simulink model "ssc_hydromech_power_split_cvt_engine_signal_intf"  (R2025a)
settings: Solver=ode23t  StartTime=0.0  StopTime=70  RelTol=1e-3  AbsTol=1e-3
StartFcn:
  | tic
StopFcn:
  | Elapsed_Sim_Time = toc;
  | disp(['Elapsed Sim Time = ' num2str(Elapsed_Sim_Time)]);
undefined symbols (not defined in the file): DiscIntNeverNeededParam, HMPST, K, Lambda, tau, x0
libraries: fl_lib x30, nesl_utility x16, sm_wheel_loader_lib x9, simulink x7, simulink_extras x6, sdl_lib x3
(part 1 of 4)
Description:
  | Wheel Loader CVT with Signal Interface
  | Copyright 2023-2025 The MathWorks, Inc.
settings Model: TunableVars=Init_Veh_TopSpeed  TunableVarsStorageClass=Auto  Creator=Shusen Zhang  LastModifiedBy=smiller
settings SolverCC: AutoScaleAbsTol=off  MaxConsecutiveMinStep=5
settings DataIOCC: ReturnWorkspaceOutputs=off  SignalLoggingName=logsout_ssc_hydromech_power_split_cvt_engine_signal_intf
settings DebuggingCC: UnderspecifiedInitializationDetection=Classic  MergeDetectMultiDrivingBlocksExec=none
settings ModelReferenceCC: PropagateSignalLabelsOutOfModel=off
settings RTWCC: GPUComputeCapability=3.5
settings SimscapeCC: SimscapeLogType=all  SimscapeLogName=simlog_ssc_hydromech_power_split_cvt_engine_signal_intf  SimscapeLogLimitData=off
settings ExplorerConfigSet: SimMechanicsOpenEditorOnUpdate=off

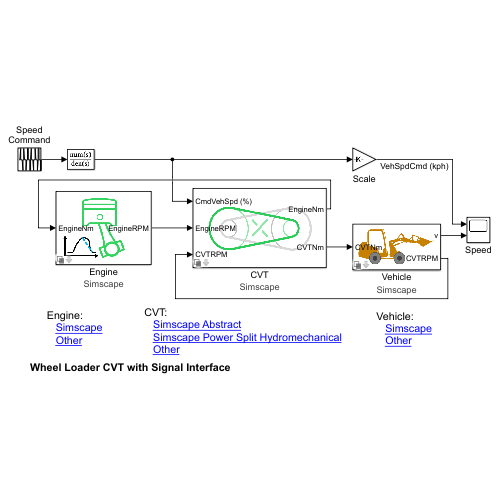
[thumbnail: Simulink's stored preview of the top-level diagram]
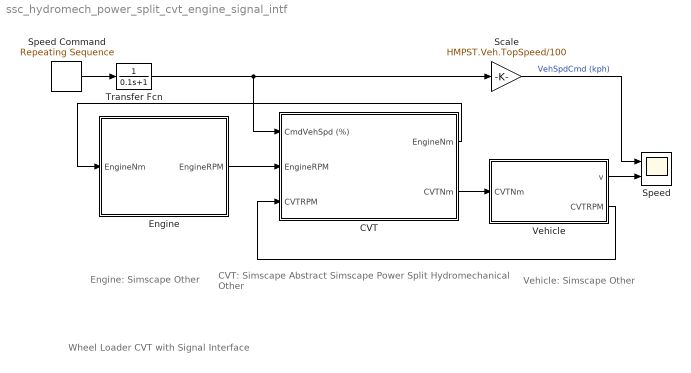
== system ssc_hydromech_power_split_cvt_engine_signal_intf ==
  note: Wheel Loader CVT with Signal Interface
  note: CVT:
      | Simscape Abstract
      | Simscape Power Split Hydromechanical
      | Other
  note: Vehicle:
      | Simscape
      | Other
  note: Engine:
      | Simscape
      | Other
  CVT : Subsystem  Variant=on  VariantControlMode=label  VariantControl=CVT  LabelModeActiveChoice=Simscape
      settings: AttributesFormatString=%<LabelModeActiveChoice>
  Engine : Subsystem  Variant=on  VariantControlMode=label  VariantControl=Engine  LabelModeActiveChoice=Simscape
      settings: AttributesFormatString=%<LabelModeActiveChoice>
  Scale : Gain  Gain=HMPST.Veh.TopSpeed/100
  Speed : Scope  NumInputPorts=2
      settings: ActiveDisplayYMinimum=-9.8692  ActiveDisplayYMaximum=9.88206
  Speed Command : simulink/Sources/Repeating Sequence  rep_seq_t=[0 10 12 15 17 32 34 37 39 41 43 46 48 63 65 68 70]  rep_seq_y=[0 0 1 1 0 0 -1 -1 0 0 1 1 0 0 -1 -1 0]*25
  Transfer Fcn : TransferFcn  Denominator=[0.1 1]
  Vehicle : Subsystem  Variant=on  VariantControlMode=label  VariantControl=Vehicle  LabelModeActiveChoice=Simscape
      settings: AttributesFormatString=%<LabelModeActiveChoice>
  wires:
  Speed Command/1 -> Transfer Fcn/1
  Transfer Fcn/1 -> Scale/1, CVT/1(CmdVehSpd (%))
  Engine/1(EngineRPM) -> CVT/2(EngineRPM)
  CVT/1(EngineNm) -> Engine/1(EngineNm)
  CVT/2(CVTNm) -> Vehicle/1(CVTNm)
  Vehicle/1(v) -> Speed/2
  Vehicle/2(CVTRPM) -> CVT/3(CVTRPM)
  Scale/1 -> Speed/1  "VehSpdCmd (kph)"

== system ssc_hydromech_power_split_cvt_engine_signal_intf/CVT ==
  CmdVehSpd (%) : Inport
  EngineRPM : Inport  Port=2
  CVTRPM : Inport  Port=3
  Other : Subsystem  VariantControl=Other
  Simscape : Subsystem  VariantControl=Simscape
      mask Display:
      | activeVar = get_param([gcb '/Transmission'],'LabelModeActiveChoice');
      | 
      | if(strcmp(activeVar,'Abstract'))
      |     image('ssc_cvt_abstract_IMAGE.png');
      | elseif(strcmp(activeVar,'Hydrostatic'))
      |     image('sm_wheel_loader_hydrostatic_IMAGE.png');
      | elseif(strcmp(activeVar,'Power_Split_HM'))
      |     image('ssc_hydromech_power_split_cvt_IMAGE.png');
      | end
  EngineNm : Outport
  CVTNm : Outport  Port=2

== system ssc_hydromech_power_split_cvt_engine_signal_intf/Engine ==
  EngineNm : Inport
  Other : Subsystem  VariantControl=Other
  Simscape : Subsystem  VariantControl=Simscape
      mask Display: image('sdl_engine_Droop_IMAGE.png')
  EngineRPM : Outport

== system ssc_hydromech_power_split_cvt_engine_signal_intf/Vehicle ==
  CVTNm : Inport
  Other : Subsystem  VariantControl=Other
  Simscape : Subsystem  VariantControl=Simscape
      mask Display: image('sm_wheel_loader_vehicle1D_IMAGE.png');
  v : Outport
  CVTRPM : Outport  Port=2

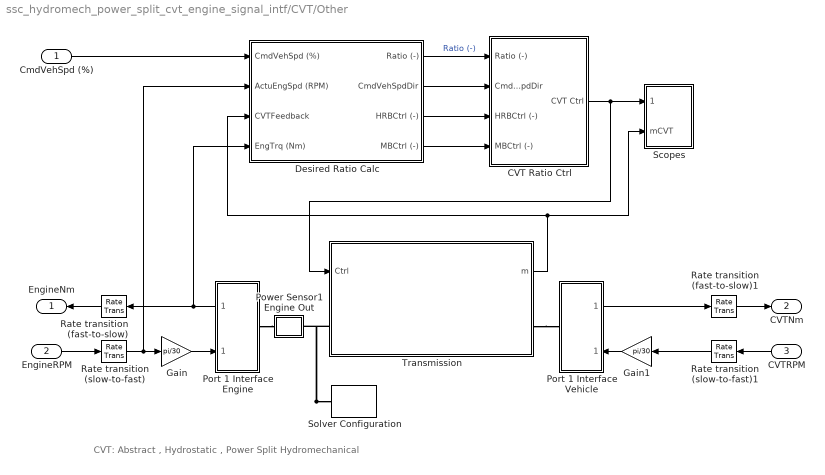
== system ssc_hydromech_power_split_cvt_engine_signal_intf/CVT/Other ==
  note: CVT: Abstract , Hydrostatic , Power Split Hydromechanical
  CmdVehSpd (%) : Inport
  EngineRPM : Inport  Port=2
  CVTRPM : Inport  Port=3
  CVT Ratio Ctrl : Subsystem
  Desired Ratio Calc : Subsystem
  Gain : Gain  Gain=pi/30
  Gain1 : Gain  Gain=pi/30
  Port 1 Interface Engine : Subsystem  mask(Network Coupler (Flexible Shaft) Port 1 Interface){interfaceModel=an actual shaft compliance, k=250, lambda=20*10, samplingType=Variable step at port 1 and fixed step at port 2, ts=0.001, h1=0.001, h2=1/60, predictionDiscreteToContinuous=off, smoothingContinuousToDiscrete=off, predictionSlowToFast=off, smoothingFastToSlow=off, nSmooth=1, tsSmoothing=0.01, J1=1, J2=1, tsRecommended=0.0026611, hRecommended=0.00026611, kDerived=250, lambdaDerived=20, tsMax=0.11975, through0=0}
      mask prompts: interfaceModel "physmod:simscape:couplers:SimscapeNetworkCouplersLib:SeparateUsing_MP"; k "physmod:simscape:couplers:SimscapeNetworkCouplersLib:ShaftStiffnessNmrad_MP"; lambda "physmod:simscape:couplers:SimscapeNetworkCouplersLib:ShaftDampingNmrads_MP"; samplingType "physmod:simscape:couplers:SimscapeNetworkCouplersLib:SamplingType_MP"; ts "physmod:simscape:couplers:SimscapeNetworkCouplersLib:SeparatorTimeConstants_MP"; h1 "physmod:simscape:couplers:SimscapeNetworkCouplersLib:Port1NetworkDiscreteSampleTimes_MP"; h2 "physmod:simscape:couplers:SimscapeNetworkCouplersLib:Port2NetworkDiscreteSampleTimes_MP"; predictionDiscreteToContinuous "physmod:simscape:couplers:SimscapeNetworkCouplersLib:UsePredictionWhenConnectingFixedStepToVariableStep_MP"; smoothingContinuousToDiscrete "physmod:simscape:couplers:SimscapeNetworkCouplersLib:UseSmoothingWhenConnectingVariableStepToFixedStep_MP"; predictionSlowToFast "physmod:simscape:couplers:SimscapeNetworkCouplersLib:UsePredictionWhenConnectingSlowToFastSampleTimes_MP"; smoothingFastToSlow "physmod:simscape:couplers:SimscapeNetworkCouplersLib:UseSmoothingWhenConnectingFastToSlowSampleTimes_MP"; nSmooth "physmod:simscape:couplers:SimscapeNetworkCouplersLib:NumberOfSamplesOverWhichToSmooth_MP"; tsSmoothing "physmod:simscape:couplers:SimscapeNetworkCouplersLib:SmoothingTimeConstants_MP"; J1 "physmod:simscape:couplers:SimscapeNetworkCouplersLib:ApproximateInertiaAtPort1kgm2_MP"; J2 "physmod:simscape:couplers:SimscapeNetworkCouplersLib:ApproximateInertiaAtPort2kgm2_MP"; tsRecommended "physmod:simscape:couplers:SimscapeNetworkCouplersLib:RecommendedMaxFilterTimeConstants_MP"; hRecommended "physmod:simscape:couplers:SimscapeNetworkCouplersLib:RecommendedMaxDiscreteSampleTimes_MP"; kDerived "physmod:simscape:couplers:SimscapeNetworkCouplersLib:CalculatedShaftStiffnessNmrad_MP"; lambdaDerived "physmod:simscape:couplers:SimscapeNetworkCouplersLib:CalculatedShaftDampingNmrads_MP"; tsMax "physmod:simscape:couplers:SimscapeNetworkCouplersLib:CalculatedFastestTrackableTimeConstants_MP"; through0 "physmod:simscape:couplers:SimscapeNetworkCouplersLib:InitialTransmittedTorqueNm_MP"
      mask help: physmod:simscape:couplers:SimscapeNetworkCouplersLib:NetworkCouplerFlexibleShaftPort1Interface_MD
      mask init:
      | % Fixed step sample time value check
      | foundation.internal.couplers.checkSampleTimes(gcb,h1,h2);
      | 
      | % Map mask choices to Simscape block parameters  
      | [K,Lambda,tau,~,~,x0,~] = foundation.internal.couplers.mechanical.derivedParamsRotational(...
      |     gcb,ts,h1,h2,through0,k,lambda,J1,J2);
      settings: PortSchema="{\"entries\":[{\"content\":{\"sides\":[{\"content\":{\"connectorIds\":[\"LConn1\"]},\"type\":\"ConnectorPlacement.EquallySpacedRectSide\",\"uuid\":\"a6d4a9fd-b5aa-40dc-ab7e-2b646b9b57bc\"},{\"content\":{\"connectorIds\":[\"Out1\",\"In1\"],\"side\":\"RIGHT\"},\"type\":\"ConnectorPlacement.EquallySpacedRectSide\",\"uuid\":\"31bb6273-5b9b-48d0-a1a2-6fbacb979b97\"},{\"content\":{\"connectorIds\":[],\"side\":\"TOP\"},\"type\":\"ConnectorPlacement.EquallySpacedRectSide\",\"uuid\":\"0f7afab2-4481-486c-9ad0-2b42c5b091a4\"}]},\"type\":\"ConnectorPlacement.EquallySpacedConnector\",\"uuid\":\"a98e47aa-cbfd-441a-b14c-c9ea515c056e\"}],\"packageUris\":[\"http://schema.mathworks.com/mf0/Connector/R2020b\"],\"version\":\"1.0\"}"
      mask Help: web([docroot '/simscape/ref/networkcouplerflexibleshaft.html'])
      mask TypeOptions interfaceModel: physmod:simscape:couplers:SimscapeNetworkCouplersLib:anActualShaftCompliance_PV | physmod:simscape:couplers:SimscapeNetworkCouplersLib:anAddedNumericalCompliance_PV
      mask Callback interfaceModel: foundation.internal.couplers.mechanical.parameterVisibilities(gcb)
      mask TypeOptions samplingType: physmod:simscape:couplers:SimscapeNetworkCouplersLib:VariableStepAtPorts1And2_PV | physmod:simscape:couplers:SimscapeNetworkCouplersLib:VariableStepAtPort1AndFixedStepAtPort2_PV | physmod:simscape:couplers:SimscapeNetworkCouplersLib:FixedStepBothPortsWithCommonSampleTime_PV | physmod:simscape:couplers:SimscapeNetworkCouplersLib:FixedStepBothPortsWithFasterSamplingAtPort1_PV
      mask Callback samplingType: foundation.internal.couplers.mechanical.parameterVisibilities(gcb)
      mask Callback predictionDiscreteToContinuous: foundation.internal.couplers.mechanical.parameterVisibilities(gcb)
      mask Callback smoothingContinuousToDiscrete: foundation.internal.couplers.mechanical.parameterVisibilities(gcb)
      mask Callback predictionSlowToFast: foundation.internal.couplers.mechanical.parameterVisibilities(gcb)
      mask Callback smoothingFastToSlow: foundation.internal.couplers.mechanical.parameterVisibilities(gcb)
      mask DialogControl Main Prompt: physmod:simscape:couplers:SimscapeNetworkCouplersLib:tab_Main
      mask DialogControl interfaceModel Prompt: Separate using
      mask DialogControl k Prompt: Shaft stiffness (Nm/rad)
      mask DialogControl lambda Prompt: Shaft damping (Nm/(rad/s))
      mask DialogControl samplingType Prompt: Sampling type
      mask DialogControl ts Prompt: Separator time constant (s)
      mask DialogControl h1 Prompt: Port 1 network discrete sample time (s)
      mask DialogControl h2 Prompt: Port 2 network discrete sample time (s)
      mask DialogControl predictionDiscreteToContinuous Prompt: Use prediction when connecting fixed step to variable step
      mask DialogControl smoothingContinuousToDiscrete Prompt: Use smoothing when connecting variable step to fixed step
      mask DialogControl predictionSlowToFast Prompt: Use prediction when connecting slow to fast sample times
      mask DialogControl smoothingFastToSlow Prompt: Use smoothing when connecting fast to slow sample times
      mask DialogControl nSmooth Prompt: Number of samples over which to smooth
      mask DialogControl tsSmoothing Prompt: Smoothing time constant (s)
      mask DialogControl Analysis Prompt: physmod:simscape:couplers:SimscapeNetworkCouplersLib:tab_Analysis
      mask DialogControl connectedNetworkInfo Prompt: physmod:simscape:couplers:SimscapeNetworkCouplersLib:heading_ConnectedNetworkInformation
      mask DialogControl J1 Prompt: Approximate inertia at port 1 (kg*m^2)
      mask DialogControl J2 Prompt: Approximate inertia at port 2 (kg*m^2)
      mask DialogControl derivedValues Prompt: physmod:simscape:couplers:SimscapeNetworkCouplersLib:heading_DerivedValues
      mask DialogControl tsRecommended Prompt: Recommended max filter time constant (s)
      mask DialogControl hRecommended Prompt: Recommended max discrete sample time (s)
      mask DialogControl kDerived Prompt: Calculated shaft stiffness (Nm/rad)
      mask DialogControl lambdaDerived Prompt: Calculated shaft damping (Nm/(rad/s))
      mask DialogControl tsMax Prompt: Calculated fastest trackable time constant (s)
      mask DialogControl updateRecommendations Prompt: physmod:simscape:couplers:SimscapeNetworkCouplersLib:button_Update
      mask DialogControl updateRecommendations Callback: foundation.internal.couplers.mechanical.analysisRotational(gcb);
      mask DialogControl InitialConditions Prompt: physmod:simscape:couplers:SimscapeNetworkCouplersLib:tab_InitialConditions
      mask DialogControl through0 Prompt: Initial transmitted torque (Nm)
  Port 1 Interface Vehicle : Subsystem  mask(Network Coupler (Flexible Shaft) Port 1 Interface){interfaceModel=an actual shaft compliance, k=250*10, lambda=20*10, samplingType=Variable step at port 1 and fixed step at port 2, ts=0.001, h1=0.001, h2=1/60, predictionDiscreteToContinuous=off, smoothingContinuousToDiscrete=off, predictionSlowToFast=off, smoothingFastToSlow=off, nSmooth=1, tsSmoothing=0.01, J1=1, J2=1, tsRecommended=0.0026611, hRecommended=0.00026611, kDerived=250, lambdaDerived=20, tsMax=0.11975, through0=0}
      mask prompts: interfaceModel "physmod:simscape:couplers:SimscapeNetworkCouplersLib:SeparateUsing_MP"; k "physmod:simscape:couplers:SimscapeNetworkCouplersLib:ShaftStiffnessNmrad_MP"; lambda "physmod:simscape:couplers:SimscapeNetworkCouplersLib:ShaftDampingNmrads_MP"; samplingType "physmod:simscape:couplers:SimscapeNetworkCouplersLib:SamplingType_MP"; ts "physmod:simscape:couplers:SimscapeNetworkCouplersLib:SeparatorTimeConstants_MP"; h1 "physmod:simscape:couplers:SimscapeNetworkCouplersLib:Port1NetworkDiscreteSampleTimes_MP"; h2 "physmod:simscape:couplers:SimscapeNetworkCouplersLib:Port2NetworkDiscreteSampleTimes_MP"; predictionDiscreteToContinuous "physmod:simscape:couplers:SimscapeNetworkCouplersLib:UsePredictionWhenConnectingFixedStepToVariableStep_MP"; smoothingContinuousToDiscrete "physmod:simscape:couplers:SimscapeNetworkCouplersLib:UseSmoothingWhenConnectingVariableStepToFixedStep_MP"; predictionSlowToFast "physmod:simscape:couplers:SimscapeNetworkCouplersLib:UsePredictionWhenConnectingSlowToFastSampleTimes_MP"; smoothingFastToSlow "physmod:simscape:couplers:SimscapeNetworkCouplersLib:UseSmoothingWhenConnectingFastToSlowSampleTimes_MP"; nSmooth "physmod:simscape:couplers:SimscapeNetworkCouplersLib:NumberOfSamplesOverWhichToSmooth_MP"; tsSmoothing "physmod:simscape:couplers:SimscapeNetworkCouplersLib:SmoothingTimeConstants_MP"; J1 "physmod:simscape:couplers:SimscapeNetworkCouplersLib:ApproximateInertiaAtPort1kgm2_MP"; J2 "physmod:simscape:couplers:SimscapeNetworkCouplersLib:ApproximateInertiaAtPort2kgm2_MP"; tsRecommended "physmod:simscape:couplers:SimscapeNetworkCouplersLib:RecommendedMaxFilterTimeConstants_MP"; hRecommended "physmod:simscape:couplers:SimscapeNetworkCouplersLib:RecommendedMaxDiscreteSampleTimes_MP"; kDerived "physmod:simscape:couplers:SimscapeNetworkCouplersLib:CalculatedShaftStiffnessNmrad_MP"; lambdaDerived "physmod:simscape:couplers:SimscapeNetworkCouplersLib:CalculatedShaftDampingNmrads_MP"; tsMax "physmod:simscape:couplers:SimscapeNetworkCouplersLib:CalculatedFastestTrackableTimeConstants_MP"; through0 "physmod:simscape:couplers:SimscapeNetworkCouplersLib:InitialTransmittedTorqueNm_MP"
      mask help: physmod:simscape:couplers:SimscapeNetworkCouplersLib:NetworkCouplerFlexibleShaftPort1Interface_MD
      mask init: same as ssc_hydromech_power_split_cvt_engine_signal_intf/CVT/Other/Port 1 Interface Engine
      settings: PortSchema="{\"entries\":[{\"content\":{\"sides\":[{\"content\":{\"connectorIds\":[\"LConn1\"]},\"type\":\"ConnectorPlacement.EquallySpacedRectSide\",\"uuid\":\"a6d4a9fd-b5aa-40dc-ab7e-2b646b9b57bc\"},{\"content\":{\"connectorIds\":[\"Out1\",\"In1\"],\"side\":\"RIGHT\"},\"type\":\"ConnectorPlacement.EquallySpacedRectSide\",\"uuid\":\"31bb6273-5b9b-48d0-a1a2-6fbacb979b97\"},{\"content\":{\"connectorIds\":[],\"side\":\"TOP\"},\"type\":\"ConnectorPlacement.EquallySpacedRectSide\",\"uuid\":\"0f7afab2-4481-486c-9ad0-2b42c5b091a4\"}]},\"type\":\"ConnectorPlacement.EquallySpacedConnector\",\"uuid\":\"a98e47aa-cbfd-441a-b14c-c9ea515c056e\"}],\"packageUris\":[\"http://schema.mathworks.com/mf0/Connector/R2020b\"],\"version\":\"1.0\"}"
      mask Help: web([docroot '/simscape/ref/networkcouplerflexibleshaft.html'])
      mask TypeOptions interfaceModel: physmod:simscape:couplers:SimscapeNetworkCouplersLib:anActualShaftCompliance_PV | physmod:simscape:couplers:SimscapeNetworkCouplersLib:anAddedNumericalCompliance_PV
      mask Callback interfaceModel: foundation.internal.couplers.mechanical.parameterVisibilities(gcb)
      mask TypeOptions samplingType: physmod:simscape:couplers:SimscapeNetworkCouplersLib:VariableStepAtPorts1And2_PV | physmod:simscape:couplers:SimscapeNetworkCouplersLib:VariableStepAtPort1AndFixedStepAtPort2_PV | physmod:simscape:couplers:SimscapeNetworkCouplersLib:FixedStepBothPortsWithCommonSampleTime_PV | physmod:simscape:couplers:SimscapeNetworkCouplersLib:FixedStepBothPortsWithFasterSamplingAtPort1_PV
      mask Callback samplingType: foundation.internal.couplers.mechanical.parameterVisibilities(gcb)
      mask Callback predictionDiscreteToContinuous: foundation.internal.couplers.mechanical.parameterVisibilities(gcb)
      mask Callback smoothingContinuousToDiscrete: foundation.internal.couplers.mechanical.parameterVisibilities(gcb)
      mask Callback predictionSlowToFast: foundation.internal.couplers.mechanical.parameterVisibilities(gcb)
      mask Callback smoothingFastToSlow: foundation.internal.couplers.mechanical.parameterVisibilities(gcb)
      mask DialogControl Main Prompt: physmod:simscape:couplers:SimscapeNetworkCouplersLib:tab_Main
      mask DialogControl interfaceModel Prompt: Separate using
      mask DialogControl k Prompt: Shaft stiffness (Nm/rad)
      mask DialogControl lambda Prompt: Shaft damping (Nm/(rad/s))
      mask DialogControl samplingType Prompt: Sampling type
      mask DialogControl ts Prompt: Separator time constant (s)
      mask DialogControl h1 Prompt: Port 1 network discrete sample time (s)
      mask DialogControl h2 Prompt: Port 2 network discrete sample time (s)
      mask DialogControl predictionDiscreteToContinuous Prompt: Use prediction when connecting fixed step to variable step
      mask DialogControl smoothingContinuousToDiscrete Prompt: Use smoothing when connecting variable step to fixed step
      mask DialogControl predictionSlowToFast Prompt: Use prediction when connecting slow to fast sample times
      mask DialogControl smoothingFastToSlow Prompt: Use smoothing when connecting fast to slow sample times
      mask DialogControl nSmooth Prompt: Number of samples over which to smooth
      mask DialogControl tsSmoothing Prompt: Smoothing time constant (s)
      mask DialogControl Analysis Prompt: physmod:simscape:couplers:SimscapeNetworkCouplersLib:tab_Analysis
      mask DialogControl connectedNetworkInfo Prompt: physmod:simscape:couplers:SimscapeNetworkCouplersLib:heading_ConnectedNetworkInformation
      mask DialogControl J1 Prompt: Approximate inertia at port 1 (kg*m^2)
      mask DialogControl J2 Prompt: Approximate inertia at port 2 (kg*m^2)
      mask DialogControl derivedValues Prompt: physmod:simscape:couplers:SimscapeNetworkCouplersLib:heading_DerivedValues
      mask DialogControl tsRecommended Prompt: Recommended max filter time constant (s)
      mask DialogControl hRecommended Prompt: Recommended max discrete sample time (s)
      mask DialogControl kDerived Prompt: Calculated shaft stiffness (Nm/rad)
      mask DialogControl lambdaDerived Prompt: Calculated shaft damping (Nm/(rad/s))
      mask DialogControl tsMax Prompt: Calculated fastest trackable time constant (s)
      mask DialogControl updateRecommendations Prompt: physmod:simscape:couplers:SimscapeNetworkCouplersLib:button_Update
      mask DialogControl updateRecommendations Callback: foundation.internal.couplers.mechanical.analysisRotational(gcb);
      mask DialogControl InitialConditions Prompt: physmod:simscape:couplers:SimscapeNetworkCouplersLib:tab_InitialConditions
      mask DialogControl through0 Prompt: Initial transmitted torque (Nm)
  Power Sensor1 Engine Out : Subsystem
  Rate transition (fast-to-slow) : RateTransition  Integrity=off
  Rate transition (fast-to-slow)1 : RateTransition  Integrity=off
  Rate transition (slow-to-fast) : RateTransition  Integrity=off
  Rate transition (slow-to-fast)1 : RateTransition  Integrity=off
  Scopes : Subsystem
  Solver Configuration : nesl_utility/Solver Configuration  PhysicalDomain=network_engine_domain  SubClassName=solver  LeftPortType=input  RightPortType=generic  Tones=[]  Harmonics=[]  SimulateNoise=off  Profile=off  UseLocalSampling=off  EnableSwitchedLinearOptims=on  FrequencyDomain=off  UseCCode=off  RelTol=0.001  AbsTol=1e-06  MinStep=1e-09  ToWorkspace=off  RevertToSquareIcSolve=off  NumHomotopyIterations=100  PhasorMode=off  PhasorModeNumHarmonics=1  ConsistencySolver=NEWTON_XTOL_AFTER_FTOL  IndexReductionMethod=DerivativeReplacement  DoDC=off  ResidualTolerance=1e-09  ConsistencyTolSource=GLOBAL  ConsistencyAbsTol=0.001  ConsistencyRelTol=0.001  ConsistencyTolFactor=0.001  UseLocalSolver=off  LocalSolverChoice=NE_BACKWARD_EULER_ADVANCER  ResolveIndetEquations=on  FunctionEvalNumThread=1  LocalSolverSampleTime=0.001  DoFixedCost=off  MaxNonlinIter=1  MaxModeIter=2  ComputeImpulses=off  ImpulseIterations=2  LinearAlgebra=Sparse  LinearAlgebraNumThread=0  EquationFormulation=NE_TIME_EF  DelaysMemoryBudget=1024  AutomaticFiltering=on  FilteringTimeConstant=0.001  PartitionStorageMethod=AS_NEEDED  PartitionMemoryBudget=1024  PartitionMethod=FAST  MultibodyUseLocalSolver=off  MultibodyLocalSolverChoice=ODE1  MultibodyLocalSolverSampleTime=0.001
  Transmission : Subsystem  Variant=on  VariantControlMode=label  VariantControl=Choice  LabelModeActiveChoice=Abstract
      settings: AttributesFormatString=%<LabelModeActiveChoice>
  EngineNm : Outport
  CVTNm : Outport  Port=2
  wires:
  Transmission/1(m) -> Desired Ratio Calc/3(CVTFeedback), Scopes/2(mCVT)
  CVT Ratio Ctrl/1(CVT Ctrl) -> Scopes/1(CVTCtrl), Transmission/1(Ctrl)
  EngineRPM/1 -> Rate transition (slow-to-fast)/1
  Rate transition (slow-to-fast)1/1 -> Gain1/1
  Port 1 Interface Vehicle/1(torque) -> Rate transition (fast-to-slow)1/1
  CVTRPM/1 -> Rate transition (slow-to-fast)1/1
  Gain/1 -> Port 1 Interface Engine/1(speed)
  Gain1/1 -> Port 1 Interface Vehicle/1(speed)
  Rate transition (fast-to-slow)1/1 -> CVTNm/1
  Rate transition (fast-to-slow)/1 -> EngineNm/1
  CmdVehSpd (%)/1 -> Desired Ratio Calc/1(CmdVehSpd (%))
  Desired Ratio Calc/4(MBCtrl (-)) -> CVT Ratio Ctrl/4(MBCtrl (-))
  Rate transition (slow-to-fast)/1 -> Gain/1, Desired Ratio Calc/2(ActuEngSpd (RPM))
  Port 1 Interface Engine/1(torque) -> Rate transition (fast-to-slow)/1, Desired Ratio Calc/4(EngTrq (Nm))
  Desired Ratio Calc/1(Ratio (-)) -> CVT Ratio Ctrl/1(Ratio (-))  "Ratio (-)"
  Desired Ratio Calc/2(CmdVehSpdDir) -> CVT Ratio Ctrl/2(CmdVehSpdDir)
  Desired Ratio Calc/3(HRBCtrl (-)) -> CVT Ratio Ctrl/3(HRBCtrl (-))
  connections:
  Solver Configuration/RConn1 -- Transmission/LConn1 -- Power Sensor1 Engine Out/RConn1
  Port 1 Interface Engine/LConn1 -- Power Sensor1 Engine Out/LConn1
  Transmission/RConn1 -- Port 1 Interface Vehicle/LConn1

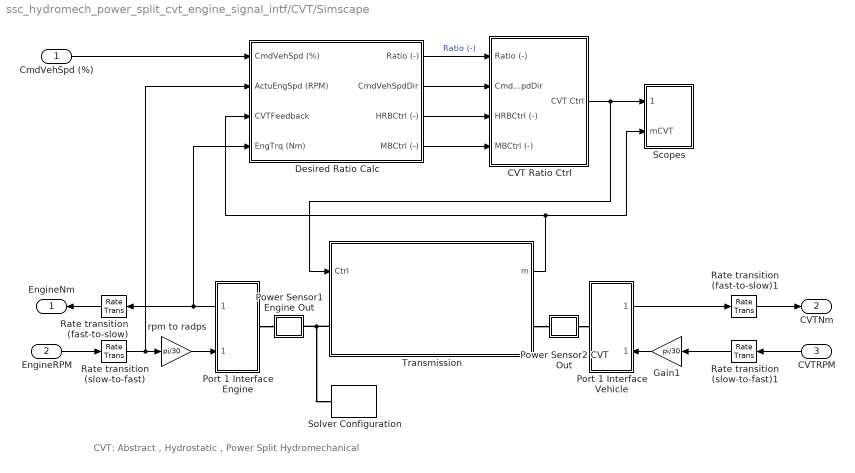
== system ssc_hydromech_power_split_cvt_engine_signal_intf/CVT/Simscape ==
  note: CVT: Abstract , Hydrostatic , Power Split Hydromechanical
  CmdVehSpd (%) : Inport
  EngineRPM : Inport  Port=2
  CVTRPM : Inport  Port=3
  CVT Ratio Ctrl : Subsystem
  Desired Ratio Calc : Subsystem
  Gain1 : Gain  Gain=pi/30
  Port 1 Interface Engine : Subsystem  mask(Network Coupler (Flexible Shaft) Port 1 Interface){interfaceModel=an actual shaft compliance, k=250, lambda=20*10, samplingType=Variable step at port 1 and fixed step at port 2, ts=0.001, h1=0.001, h2=1/60, predictionDiscreteToContinuous=off, smoothingContinuousToDiscrete=off, predictionSlowToFast=off, smoothingFastToSlow=off, nSmooth=1, tsSmoothing=0.01, J1=1, J2=1, tsRecommended=0.0026611, hRecommended=0.00026611, kDerived=250, lambdaDerived=20, tsMax=0.11975, through0=70}
      mask prompts: interfaceModel "physmod:simscape:couplers:SimscapeNetworkCouplersLib:SeparateUsing_MP"; k "physmod:simscape:couplers:SimscapeNetworkCouplersLib:ShaftStiffnessNmrad_MP"; lambda "physmod:simscape:couplers:SimscapeNetworkCouplersLib:ShaftDampingNmrads_MP"; samplingType "physmod:simscape:couplers:SimscapeNetworkCouplersLib:SamplingType_MP"; ts "physmod:simscape:couplers:SimscapeNetworkCouplersLib:SeparatorTimeConstants_MP"; h1 "physmod:simscape:couplers:SimscapeNetworkCouplersLib:Port1NetworkDiscreteSampleTimes_MP"; h2 "physmod:simscape:couplers:SimscapeNetworkCouplersLib:Port2NetworkDiscreteSampleTimes_MP"; predictionDiscreteToContinuous "physmod:simscape:couplers:SimscapeNetworkCouplersLib:UsePredictionWhenConnectingFixedStepToVariableStep_MP"; smoothingContinuousToDiscrete "physmod:simscape:couplers:SimscapeNetworkCouplersLib:UseSmoothingWhenConnectingVariableStepToFixedStep_MP"; predictionSlowToFast "physmod:simscape:couplers:SimscapeNetworkCouplersLib:UsePredictionWhenConnectingSlowToFastSampleTimes_MP"; smoothingFastToSlow "physmod:simscape:couplers:SimscapeNetworkCouplersLib:UseSmoothingWhenConnectingFastToSlowSampleTimes_MP"; nSmooth "physmod:simscape:couplers:SimscapeNetworkCouplersLib:NumberOfSamplesOverWhichToSmooth_MP"; tsSmoothing "physmod:simscape:couplers:SimscapeNetworkCouplersLib:SmoothingTimeConstants_MP"; J1 "physmod:simscape:couplers:SimscapeNetworkCouplersLib:ApproximateInertiaAtPort1kgm2_MP"; J2 "physmod:simscape:couplers:SimscapeNetworkCouplersLib:ApproximateInertiaAtPort2kgm2_MP"; tsRecommended "physmod:simscape:couplers:SimscapeNetworkCouplersLib:RecommendedMaxFilterTimeConstants_MP"; hRecommended "physmod:simscape:couplers:SimscapeNetworkCouplersLib:RecommendedMaxDiscreteSampleTimes_MP"; kDerived "physmod:simscape:couplers:SimscapeNetworkCouplersLib:CalculatedShaftStiffnessNmrad_MP"; lambdaDerived "physmod:simscape:couplers:SimscapeNetworkCouplersLib:CalculatedShaftDampingNmrads_MP"; tsMax "physmod:simscape:couplers:SimscapeNetworkCouplersLib:CalculatedFastestTrackableTimeConstants_MP"; through0 "physmod:simscape:couplers:SimscapeNetworkCouplersLib:InitialTransmittedTorqueNm_MP"
      mask help: physmod:simscape:couplers:SimscapeNetworkCouplersLib:NetworkCouplerFlexibleShaftPort1Interface_MD
      mask init: same as ssc_hydromech_power_split_cvt_engine_signal_intf/CVT/Other/Port 1 Interface Engine
      settings: PortSchema="{\"entries\":[{\"content\":{\"sides\":[{\"content\":{\"connectorIds\":[\"LConn1\"]},\"type\":\"ConnectorPlacement.EquallySpacedRectSide\",\"uuid\":\"a6d4a9fd-b5aa-40dc-ab7e-2b646b9b57bc\"},{\"content\":{\"connectorIds\":[\"Out1\",\"In1\"],\"side\":\"RIGHT\"},\"type\":\"ConnectorPlacement.EquallySpacedRectSide\",\"uuid\":\"31bb6273-5b9b-48d0-a1a2-6fbacb979b97\"},{\"content\":{\"connectorIds\":[],\"side\":\"TOP\"},\"type\":\"ConnectorPlacement.EquallySpacedRectSide\",\"uuid\":\"0f7afab2-4481-486c-9ad0-2b42c5b091a4\"}]},\"type\":\"ConnectorPlacement.EquallySpacedConnector\",\"uuid\":\"a98e47aa-cbfd-441a-b14c-c9ea515c056e\"}],\"packageUris\":[\"http://schema.mathworks.com/mf0/Connector/R2020b\"],\"version\":\"1.0\"}"
      mask Help: web([docroot '/simscape/ref/networkcouplerflexibleshaft.html'])
      mask TypeOptions interfaceModel: physmod:simscape:couplers:SimscapeNetworkCouplersLib:anActualShaftCompliance_PV | physmod:simscape:couplers:SimscapeNetworkCouplersLib:anAddedNumericalCompliance_PV
      mask Callback interfaceModel: foundation.internal.couplers.mechanical.parameterVisibilities(gcb)
      mask TypeOptions samplingType: physmod:simscape:couplers:SimscapeNetworkCouplersLib:VariableStepAtPorts1And2_PV | physmod:simscape:couplers:SimscapeNetworkCouplersLib:VariableStepAtPort1AndFixedStepAtPort2_PV | physmod:simscape:couplers:SimscapeNetworkCouplersLib:FixedStepBothPortsWithCommonSampleTime_PV | physmod:simscape:couplers:SimscapeNetworkCouplersLib:FixedStepBothPortsWithFasterSamplingAtPort1_PV
      mask Callback samplingType: foundation.internal.couplers.mechanical.parameterVisibilities(gcb)
      mask Callback predictionDiscreteToContinuous: foundation.internal.couplers.mechanical.parameterVisibilities(gcb)
      mask Callback smoothingContinuousToDiscrete: foundation.internal.couplers.mechanical.parameterVisibilities(gcb)
      mask Callback predictionSlowToFast: foundation.internal.couplers.mechanical.parameterVisibilities(gcb)
      mask Callback smoothingFastToSlow: foundation.internal.couplers.mechanical.parameterVisibilities(gcb)
      mask DialogControl Main Prompt: physmod:simscape:couplers:SimscapeNetworkCouplersLib:tab_Main
      mask DialogControl interfaceModel Prompt: Separate using
      mask DialogControl k Prompt: Shaft stiffness (Nm/rad)
      mask DialogControl lambda Prompt: Shaft damping (Nm/(rad/s))
      mask DialogControl samplingType Prompt: Sampling type
      mask DialogControl ts Prompt: Separator time constant (s)
      mask DialogControl h1 Prompt: Port 1 network discrete sample time (s)
      mask DialogControl h2 Prompt: Port 2 network discrete sample time (s)
      mask DialogControl predictionDiscreteToContinuous Prompt: Use prediction when connecting fixed step to variable step
      mask DialogControl smoothingContinuousToDiscrete Prompt: Use smoothing when connecting variable step to fixed step
      mask DialogControl predictionSlowToFast Prompt: Use prediction when connecting slow to fast sample times
      mask DialogControl smoothingFastToSlow Prompt: Use smoothing when connecting fast to slow sample times
      mask DialogControl nSmooth Prompt: Number of samples over which to smooth
      mask DialogControl tsSmoothing Prompt: Smoothing time constant (s)
      mask DialogControl Analysis Prompt: physmod:simscape:couplers:SimscapeNetworkCouplersLib:tab_Analysis
      mask DialogControl connectedNetworkInfo Prompt: physmod:simscape:couplers:SimscapeNetworkCouplersLib:heading_ConnectedNetworkInformation
      mask DialogControl J1 Prompt: Approximate inertia at port 1 (kg*m^2)
      mask DialogControl J2 Prompt: Approximate inertia at port 2 (kg*m^2)
      mask DialogControl derivedValues Prompt: physmod:simscape:couplers:SimscapeNetworkCouplersLib:heading_DerivedValues
      mask DialogControl tsRecommended Prompt: Recommended max filter time constant (s)
      mask DialogControl hRecommended Prompt: Recommended max discrete sample time (s)
      mask DialogControl kDerived Prompt: Calculated shaft stiffness (Nm/rad)
      mask DialogControl lambdaDerived Prompt: Calculated shaft damping (Nm/(rad/s))
      mask DialogControl tsMax Prompt: Calculated fastest trackable time constant (s)
      mask DialogControl updateRecommendations Prompt: physmod:simscape:couplers:SimscapeNetworkCouplersLib:button_Update
      mask DialogControl updateRecommendations Callback: foundation.internal.couplers.mechanical.analysisRotational(gcb);
      mask DialogControl InitialConditions Prompt: physmod:simscape:couplers:SimscapeNetworkCouplersLib:tab_InitialConditions
      mask DialogControl through0 Prompt: Initial transmitted torque (Nm)
  Port 1 Interface Vehicle : Subsystem  mask(Network Coupler (Flexible Shaft) Port 1 Interface){interfaceModel=an actual shaft compliance, k=250*10, lambda=20*10, samplingType=Variable step at port 1 and fixed step at port 2, ts=0.001, h1=0.001, h2=1/60, predictionDiscreteToContinuous=off, smoothingContinuousToDiscrete=off, predictionSlowToFast=off, smoothingFastToSlow=off, nSmooth=1, tsSmoothing=0.01, J1=1, J2=1, tsRecommended=0.0026611, hRecommended=0.00026611, kDerived=250, lambdaDerived=20, tsMax=0.11975, through0=0}
      mask prompts: interfaceModel "physmod:simscape:couplers:SimscapeNetworkCouplersLib:SeparateUsing_MP"; k "physmod:simscape:couplers:SimscapeNetworkCouplersLib:ShaftStiffnessNmrad_MP"; lambda "physmod:simscape:couplers:SimscapeNetworkCouplersLib:ShaftDampingNmrads_MP"; samplingType "physmod:simscape:couplers:SimscapeNetworkCouplersLib:SamplingType_MP"; ts "physmod:simscape:couplers:SimscapeNetworkCouplersLib:SeparatorTimeConstants_MP"; h1 "physmod:simscape:couplers:SimscapeNetworkCouplersLib:Port1NetworkDiscreteSampleTimes_MP"; h2 "physmod:simscape:couplers:SimscapeNetworkCouplersLib:Port2NetworkDiscreteSampleTimes_MP"; predictionDiscreteToContinuous "physmod:simscape:couplers:SimscapeNetworkCouplersLib:UsePredictionWhenConnectingFixedStepToVariableStep_MP"; smoothingContinuousToDiscrete "physmod:simscape:couplers:SimscapeNetworkCouplersLib:UseSmoothingWhenConnectingVariableStepToFixedStep_MP"; predictionSlowToFast "physmod:simscape:couplers:SimscapeNetworkCouplersLib:UsePredictionWhenConnectingSlowToFastSampleTimes_MP"; smoothingFastToSlow "physmod:simscape:couplers:SimscapeNetworkCouplersLib:UseSmoothingWhenConnectingFastToSlowSampleTimes_MP"; nSmooth "physmod:simscape:couplers:SimscapeNetworkCouplersLib:NumberOfSamplesOverWhichToSmooth_MP"; tsSmoothing "physmod:simscape:couplers:SimscapeNetworkCouplersLib:SmoothingTimeConstants_MP"; J1 "physmod:simscape:couplers:SimscapeNetworkCouplersLib:ApproximateInertiaAtPort1kgm2_MP"; J2 "physmod:simscape:couplers:SimscapeNetworkCouplersLib:ApproximateInertiaAtPort2kgm2_MP"; tsRecommended "physmod:simscape:couplers:SimscapeNetworkCouplersLib:RecommendedMaxFilterTimeConstants_MP"; hRecommended "physmod:simscape:couplers:SimscapeNetworkCouplersLib:RecommendedMaxDiscreteSampleTimes_MP"; kDerived "physmod:simscape:couplers:SimscapeNetworkCouplersLib:CalculatedShaftStiffnessNmrad_MP"; lambdaDerived "physmod:simscape:couplers:SimscapeNetworkCouplersLib:CalculatedShaftDampingNmrads_MP"; tsMax "physmod:simscape:couplers:SimscapeNetworkCouplersLib:CalculatedFastestTrackableTimeConstants_MP"; through0 "physmod:simscape:couplers:SimscapeNetworkCouplersLib:InitialTransmittedTorqueNm_MP"
      mask help: physmod:simscape:couplers:SimscapeNetworkCouplersLib:NetworkCouplerFlexibleShaftPort1Interface_MD
      mask init: same as ssc_hydromech_power_split_cvt_engine_signal_intf/CVT/Other/Port 1 Interface Engine
      settings: PortSchema="{\"entries\":[{\"content\":{\"sides\":[{\"content\":{\"connectorIds\":[\"LConn1\"]},\"type\":\"ConnectorPlacement.EquallySpacedRectSide\",\"uuid\":\"a6d4a9fd-b5aa-40dc-ab7e-2b646b9b57bc\"},{\"content\":{\"connectorIds\":[\"Out1\",\"In1\"],\"side\":\"RIGHT\"},\"type\":\"ConnectorPlacement.EquallySpacedRectSide\",\"uuid\":\"31bb6273-5b9b-48d0-a1a2-6fbacb979b97\"},{\"content\":{\"connectorIds\":[],\"side\":\"TOP\"},\"type\":\"ConnectorPlacement.EquallySpacedRectSide\",\"uuid\":\"0f7afab2-4481-486c-9ad0-2b42c5b091a4\"}]},\"type\":\"ConnectorPlacement.EquallySpacedConnector\",\"uuid\":\"a98e47aa-cbfd-441a-b14c-c9ea515c056e\"}],\"packageUris\":[\"http://schema.mathworks.com/mf0/Connector/R2020b\"],\"version\":\"1.0\"}"
      mask Help: web([docroot '/simscape/ref/networkcouplerflexibleshaft.html'])
      mask TypeOptions interfaceModel: physmod:simscape:couplers:SimscapeNetworkCouplersLib:anActualShaftCompliance_PV | physmod:simscape:couplers:SimscapeNetworkCouplersLib:anAddedNumericalCompliance_PV
      mask Callback interfaceModel: foundation.internal.couplers.mechanical.parameterVisibilities(gcb)
      mask TypeOptions samplingType: physmod:simscape:couplers:SimscapeNetworkCouplersLib:VariableStepAtPorts1And2_PV | physmod:simscape:couplers:SimscapeNetworkCouplersLib:VariableStepAtPort1AndFixedStepAtPort2_PV | physmod:simscape:couplers:SimscapeNetworkCouplersLib:FixedStepBothPortsWithCommonSampleTime_PV | physmod:simscape:couplers:SimscapeNetworkCouplersLib:FixedStepBothPortsWithFasterSamplingAtPort1_PV
      mask Callback samplingType: foundation.internal.couplers.mechanical.parameterVisibilities(gcb)
      mask Callback predictionDiscreteToContinuous: foundation.internal.couplers.mechanical.parameterVisibilities(gcb)
      mask Callback smoothingContinuousToDiscrete: foundation.internal.couplers.mechanical.parameterVisibilities(gcb)
      mask Callback predictionSlowToFast: foundation.internal.couplers.mechanical.parameterVisibilities(gcb)
      mask Callback smoothingFastToSlow: foundation.internal.couplers.mechanical.parameterVisibilities(gcb)
      mask DialogControl Main Prompt: physmod:simscape:couplers:SimscapeNetworkCouplersLib:tab_Main
      mask DialogControl interfaceModel Prompt: Separate using
      mask DialogControl k Prompt: Shaft stiffness (Nm/rad)
      mask DialogControl lambda Prompt: Shaft damping (Nm/(rad/s))
      mask DialogControl samplingType Prompt: Sampling type
      mask DialogControl ts Prompt: Separator time constant (s)
      mask DialogControl h1 Prompt: Port 1 network discrete sample time (s)
      mask DialogControl h2 Prompt: Port 2 network discrete sample time (s)
      mask DialogControl predictionDiscreteToContinuous Prompt: Use prediction when connecting fixed step to variable step
      mask DialogControl smoothingContinuousToDiscrete Prompt: Use smoothing when connecting variable step to fixed step
      mask DialogControl predictionSlowToFast Prompt: Use prediction when connecting slow to fast sample times
      mask DialogControl smoothingFastToSlow Prompt: Use smoothing when connecting fast to slow sample times
      mask DialogControl nSmooth Prompt: Number of samples over which to smooth
      mask DialogControl tsSmoothing Prompt: Smoothing time constant (s)
      mask DialogControl Analysis Prompt: physmod:simscape:couplers:SimscapeNetworkCouplersLib:tab_Analysis
      mask DialogControl connectedNetworkInfo Prompt: physmod:simscape:couplers:SimscapeNetworkCouplersLib:heading_ConnectedNetworkInformation
      mask DialogControl J1 Prompt: Approximate inertia at port 1 (kg*m^2)
      mask DialogControl J2 Prompt: Approximate inertia at port 2 (kg*m^2)
      mask DialogControl derivedValues Prompt: physmod:simscape:couplers:SimscapeNetworkCouplersLib:heading_DerivedValues
      mask DialogControl tsRecommended Prompt: Recommended max filter time constant (s)
      mask DialogControl hRecommended Prompt: Recommended max discrete sample time (s)
      mask DialogControl kDerived Prompt: Calculated shaft stiffness (Nm/rad)
      mask DialogControl lambdaDerived Prompt: Calculated shaft damping (Nm/(rad/s))
      mask DialogControl tsMax Prompt: Calculated fastest trackable time constant (s)
      mask DialogControl updateRecommendations Prompt: physmod:simscape:couplers:SimscapeNetworkCouplersLib:button_Update
      mask DialogControl updateRecommendations Callback: foundation.internal.couplers.mechanical.analysisRotational(gcb);
      mask DialogControl InitialConditions Prompt: physmod:simscape:couplers:SimscapeNetworkCouplersLib:tab_InitialConditions
      mask DialogControl through0 Prompt: Initial transmitted torque (Nm)
  Power Sensor1 Engine Out : Subsystem
  Power Sensor2 CVT Out : Subsystem
  Rate transition (fast-to-slow) : RateTransition  Integrity=off
  Rate transition (fast-to-slow)1 : RateTransition  Integrity=off
  Rate transition (slow-to-fast) : RateTransition  Integrity=off
  Rate transition (slow-to-fast)1 : RateTransition  Integrity=off
  Scopes : Subsystem
  Solver Configuration : nesl_utility/Solver Configuration  PhysicalDomain=network_engine_domain  SubClassName=solver  LeftPortType=input  RightPortType=generic  Tones=[]  Harmonics=[]  SimulateNoise=off  Profile=off  UseLocalSampling=off  EnableSwitchedLinearOptims=on  FrequencyDomain=off  UseCCode=off  RelTol=0.001  AbsTol=1e-06  MinStep=1e-09  ToWorkspace=off  RevertToSquareIcSolve=off  NumHomotopyIterations=100  PhasorMode=off  PhasorModeNumHarmonics=1  ConsistencySolver=NEWTON_XTOL_AFTER_FTOL  IndexReductionMethod=DerivativeReplacement  DoDC=off  ResidualTolerance=1e-09  ConsistencyTolSource=GLOBAL  ConsistencyAbsTol=0.001  ConsistencyRelTol=0.001  ConsistencyTolFactor=0.001  UseLocalSolver=off  LocalSolverChoice=NE_BACKWARD_EULER_ADVANCER  ResolveIndetEquations=on  FunctionEvalNumThread=1  LocalSolverSampleTime=0.001  DoFixedCost=off  MaxNonlinIter=1  MaxModeIter=2  ComputeImpulses=off  ImpulseIterations=2  LinearAlgebra=Sparse  LinearAlgebraNumThread=0  EquationFormulation=NE_TIME_EF  DelaysMemoryBudget=1024  AutomaticFiltering=on  FilteringTimeConstant=0.001  PartitionStorageMethod=AS_NEEDED  PartitionMemoryBudget=1024  PartitionMethod=FAST  MultibodyUseLocalSolver=off  MultibodyLocalSolverChoice=ODE1  MultibodyLocalSolverSampleTime=0.001
  Transmission : Subsystem  Variant=on  VariantControlMode=label  VariantControl=Choice  LabelModeActiveChoice=Abstract
      settings: AttributesFormatString=%<LabelModeActiveChoice>
  rpm to radps : Gain  Gain=pi/30
  EngineNm : Outport
  CVTNm : Outport  Port=2
  wires:
  Desired Ratio Calc/3(HRBCtrl (-)) -> CVT Ratio Ctrl/3(HRBCtrl (-))
  Desired Ratio Calc/2(CmdVehSpdDir) -> CVT Ratio Ctrl/2(CmdVehSpdDir)
  Desired Ratio Calc/1(Ratio (-)) -> CVT Ratio Ctrl/1(Ratio (-))  "Ratio (-)"
  Port 1 Interface Engine/1(torque) -> Desired Ratio Calc/4(EngTrq (Nm)), Rate transition (fast-to-slow)/1
  Rate transition (slow-to-fast)/1 -> Desired Ratio Calc/2(ActuEngSpd (RPM)), rpm to radps/1
  Desired Ratio Calc/4(MBCtrl (-)) -> CVT Ratio Ctrl/4(MBCtrl (-))
  CmdVehSpd (%)/1 -> Desired Ratio Calc/1(CmdVehSpd (%))
  Rate transition (fast-to-slow)/1 -> EngineNm/1
  Rate transition (fast-to-slow)1/1 -> CVTNm/1
  Gain1/1 -> Port 1 Interface Vehicle/1(speed)
  rpm to radps/1 -> Port 1 Interface Engine/1(speed)
  CVTRPM/1 -> Rate transition (slow-to-fast)1/1
  Port 1 Interface Vehicle/1(torque) -> Rate transition (fast-to-slow)1/1
  Rate transition (slow-to-fast)1/1 -> Gain1/1
  EngineRPM/1 -> Rate transition (slow-to-fast)/1
  CVT Ratio Ctrl/1(CVT Ctrl) -> Transmission/1(Ctrl), Scopes/1(CVTCtrl)
  Transmission/1(m) -> Scopes/2(mCVT), Desired Ratio Calc/3(CVTFeedback)
  connections:
  Transmission/RConn1 -- Power Sensor2 CVT Out/LConn1
  Port 1 Interface Engine/LConn1 -- Power Sensor1 Engine Out/LConn1
  Transmission/LConn1 -- Solver Configuration/RConn1 -- Power Sensor1 Engine Out/RConn1
  Power Sensor2 CVT Out/RConn1 -- Port 1 Interface Vehicle/LConn1

== system ssc_hydromech_power_split_cvt_engine_signal_intf/Engine/Other ==
  EngineNm : Inport
  Ground : Ground
  Terminator : Terminator
  EngineRPM : Outport
  wires:
  Ground/1 -> EngineRPM/1
  EngineNm/1 -> Terminator/1

== system ssc_hydromech_power_split_cvt_engine_signal_intf/Engine/Simscape ==
  EngineNm : Inport
  Bus Creator : BusCreator  Inputs=1
  Constant : Constant  Value=HMPST.Eng.wTarget
  Engine Droop : sm_wheel_loader_lib/Engine Droop  SystemSampleTime=-1  VariantControl=Droop  VariantActivationTime=update diagram  EmptyChoice=off  PassThrough=off  PassThroughVariantControl=(default)  EmptyChoiceVariantControl=(default)  AllowFlexibleInterface=on  Latency=0  AutoFrameSizeCalculation=off
  Port 2 Interface : Subsystem  mask(Network Coupler (Flexible Shaft) Port 2 Interface){}
      mask help: physmod:simscape:couplers:SimscapeNetworkCouplersLib:NetworkCouplerFlexibleShaftPort2Interface_MD
      settings: PortSchema="{\"entries\":[{\"content\":{\"sides\":[{\"content\":{\"connectorIds\":[\"In1\",\"Out1\"]},\"type\":\"ConnectorPlacement.EquallySpacedRectSide\",\"uuid\":\"5a4c1550-e77d-42df-bf3e-b81963920de7\"},{\"content\":{\"connectorIds\":[\"RConn1\"],\"side\":\"RIGHT\"},\"type\":\"ConnectorPlacement.EquallySpacedRectSide\",\"uuid\":\"3fd730f7-5937-4563-a365-595aaae9027b\"},{\"content\":{\"connectorIds\":[],\"side\":\"TOP\"},\"type\":\"ConnectorPlacement.EquallySpacedRectSide\",\"uuid\":\"c16e04e4-26e8-4fd6-98d3-59adbef44c0d\"}]},\"type\":\"ConnectorPlacement.EquallySpacedConnector\",\"uuid\":\"5588d8d0-d459-45fe-a303-1ca6654e99d0\"}],\"packageUris\":[\"http://schema.mathworks.com/mf0/Connector/R2020b\"],\"version\":\"1.0\"}"
      mask Help: web([docroot '/simscape/ref/networkcouplerflexibleshaft.html'])
  Solver Configuration : nesl_utility/Solver Configuration  PhysicalDomain=network_engine_domain  SubClassName=solver  LeftPortType=input  RightPortType=generic  Tones=[]  Harmonics=[]  SimulateNoise=off  Profile=off  UseLocalSampling=off  EnableSwitchedLinearOptims=on  FrequencyDomain=off  UseCCode=off  RelTol=0.001  AbsTol=1e-06  MinStep=1e-09  ToWorkspace=off  RevertToSquareIcSolve=off  NumHomotopyIterations=100  PhasorMode=off  PhasorModeNumHarmonics=1  ConsistencySolver=NEWTON_XTOL_AFTER_FTOL  IndexReductionMethod=DerivativeReplacement  DoDC=off  ResidualTolerance=1e-09  ConsistencyTolSource=GLOBAL  ConsistencyAbsTol=0.001  ConsistencyRelTol=0.001  ConsistencyTolFactor=0.001  UseLocalSolver=on  LocalSolverChoice=NE_BACKWARD_EULER_ADVANCER  ResolveIndetEquations=on  FunctionEvalNumThread=1  LocalSolverSampleTime=1/60  DoFixedCost=on  MaxNonlinIter=3  MaxModeIter=2  ComputeImpulses=off  ImpulseIterations=2  LinearAlgebra=Sparse  LinearAlgebraNumThread=0  EquationFormulation=NE_TIME_EF  DelaysMemoryBudget=1024  AutomaticFiltering=on  FilteringTimeConstant=0.001  PartitionStorageMethod=AS_NEEDED  PartitionMemoryBudget=1024  PartitionMethod=FAST  MultibodyUseLocalSolver=off  MultibodyLocalSolverChoice=ODE1  MultibodyLocalSolverSampleTime=0.001
      settings: AttributesFormatString=Local Solver: %<UseLocalSolver>
  Terminator : Terminator
  Terminator1 : Terminator
  EngineRPM : Outport
  wires:
  Bus Creator/1 -> Engine Droop/1
  EngineNm/1 -> Port 2 Interface/1(torque)
  Engine Droop/1 -> Terminator/1
  Port 2 Interface/1(speed) -> EngineRPM/1
  Engine Droop/2 -> Terminator1/1
  Constant/1 -> Bus Creator/1  "CmdEngSpd(RPM)"
  connections:
  Port 2 Interface/RConn1 -- Engine Droop/RConn1 -- Solver Configuration/RConn1

== system ssc_hydromech_power_split_cvt_engine_signal_intf/Vehicle/Other ==
  CVTNm : Inport
  Ground : Ground
  Ground1 : Ground
  Terminator : Terminator
  v : Outport
  CVTRPM : Outport  Port=2
  wires:
  CVTNm/1 -> Terminator/1
  Ground/1 -> v/1
  Ground1/1 -> CVTRPM/1

== system ssc_hydromech_power_split_cvt_engine_signal_intf/Vehicle/Simscape ==
  CVTNm : Inport
  Port 2 Interface Vehicle : Subsystem  mask(Network Coupler (Flexible Shaft) Port 2 Interface){}
      mask help: physmod:simscape:couplers:SimscapeNetworkCouplersLib:NetworkCouplerFlexibleShaftPort2Interface_MD
      settings: PortSchema="{\"entries\":[{\"content\":{\"sides\":[{\"content\":{\"connectorIds\":[\"In1\",\"Out1\"]},\"type\":\"ConnectorPlacement.EquallySpacedRectSide\",\"uuid\":\"5a4c1550-e77d-42df-bf3e-b81963920de7\"},{\"content\":{\"connectorIds\":[\"RConn1\"],\"side\":\"RIGHT\"},\"type\":\"ConnectorPlacement.EquallySpacedRectSide\",\"uuid\":\"3fd730f7-5937-4563-a365-595aaae9027b\"},{\"content\":{\"connectorIds\":[],\"side\":\"TOP\"},\"type\":\"ConnectorPlacement.EquallySpacedRectSide\",\"uuid\":\"c16e04e4-26e8-4fd6-98d3-59adbef44c0d\"}]},\"type\":\"ConnectorPlacement.EquallySpacedConnector\",\"uuid\":\"5588d8d0-d459-45fe-a303-1ca6654e99d0\"}],\"packageUris\":[\"http://schema.mathworks.com/mf0/Connector/R2020b\"],\"version\":\"1.0\"}"
      mask Help: web([docroot '/simscape/ref/networkcouplerflexibleshaft.html'])
  Solver Configuration : nesl_utility/Solver Configuration  PhysicalDomain=network_engine_domain  SubClassName=solver  LeftPortType=input  RightPortType=generic  Tones=[]  Harmonics=[]  SimulateNoise=off  Profile=off  UseLocalSampling=off  EnableSwitchedLinearOptims=on  FrequencyDomain=off  UseCCode=off  RelTol=0.001  AbsTol=1e-06  MinStep=1e-09  ToWorkspace=off  RevertToSquareIcSolve=off  NumHomotopyIterations=100  PhasorMode=off  PhasorModeNumHarmonics=1  ConsistencySolver=NEWTON_XTOL_AFTER_FTOL  IndexReductionMethod=DerivativeReplacement  DoDC=off  ResidualTolerance=1e-09  ConsistencyTolSource=GLOBAL  ConsistencyAbsTol=0.001  ConsistencyRelTol=0.001  ConsistencyTolFactor=0.001  UseLocalSolver=on  LocalSolverChoice=NE_BACKWARD_EULER_ADVANCER  ResolveIndetEquations=on  FunctionEvalNumThread=1  LocalSolverSampleTime=1/60  DoFixedCost=on  MaxNonlinIter=3  MaxModeIter=2  ComputeImpulses=off  ImpulseIterations=2  LinearAlgebra=Sparse  LinearAlgebraNumThread=0  EquationFormulation=NE_TIME_EF  DelaysMemoryBudget=1024  AutomaticFiltering=on  FilteringTimeConstant=0.001  PartitionStorageMethod=AS_NEEDED  PartitionMemoryBudget=1024  PartitionMethod=FAST  MultibodyUseLocalSolver=off  MultibodyLocalSolverChoice=ODE1  MultibodyLocalSolverSampleTime=0.001
      settings: AttributesFormatString=Local Solver: %<UseLocalSolver>
  Vehicle : Subsystem
      mask Display: image('sm_wheel_loader_vehicle1D_IMAGE.png');
  v : Outport
  CVTRPM : Outport  Port=2
  wires:
  Port 2 Interface Vehicle/1(speed) -> CVTRPM/1
  Vehicle/1(v) -> v/1
  CVTNm/1 -> Port 2 Interface Vehicle/1(torque)
  connections:
  Solver Configuration/RConn1 -- Vehicle/LConn1 -- Port 2 Interface Vehicle/RConn1
